simulink library "ASEToolBox2023a"  (R2023a)
settings: Solver=ode45  StartTime=0.0  StopTime=10.0  RelTol=1e-3  EnableMultiTasking=on
values from neighbouring files (symbols this model uses):
  dt = get_param(gcbh, 'g_output_datatype')    [maskSysComCallbacks_Receive.m]    (also in maskSysComCallbacks_Send.m = get_param(gcbh, 'g_input_datatype'))
undefined symbols (not defined in the file or in its folder): dCx, dCy, dCz, DiscIntNeverNeededParam, Discrete, dmassX, dmassY, dmassZ, dMx, dMy, dMz, dp, dp0, dp1, dp2, dp3, lmd_high, lmd_low, magnitude, Newton, p0, p1, p2, p3, p4, phi0, phi000, phi1, phi2, phi3, phi4, r1, r2, r3, r4, Raphson, theta0, theta1, theta2, theta3, theta4, Time, u0, u1, u2, u3, v0, v0_max, v0_min, v1, v111, v2, v222, v3, v333, v4, W1, w1, w2, W2 ... (+2)
libraries: simulink x38, etargetslib x28, simulink_extras x5, slpidlib x2, ctrlSharedLib x2, aerolibatmos2 x1, aerolibconvert2 x1, aerolibtransform2 x1, sharedtransform x1, dspstat3 x1, dspsolvers x1
(part 6 of 6)

== matlab function ASEToolBox2023a/Subsystem/Formation-Control/Consistent formation control /一致性控制——F1/Subsystem1/MATLAB Function ==
  data: i input; wx output; dt input; wy output
function [wx,wy] = w_error(i,dt)
%W_ERROR 此处显示有关此函数的摘要
%   此处显示详细说明
wx = 0.1*(cos(i*dt+pi/6)+cos(i*dt/3+pi/6)+cos(i*dt/5+pi/6)+cos(i*dt/7+pi/6));
wy = 0.1*(sin(i*dt+pi/6)+sin(i*dt/3+pi/6)+sin(i*dt/5+pi/6)+sin(i*dt/7+pi/6));

end

== matlab function ASEToolBox2023a/Subsystem/Formation-Control/Consistent formation control /一致性控制——F2/Subsystem2/MATLAB Function ==
  data: i input; wx output; dt input; wy output
function [wx,wy] = w_error(i,dt)
%W_ERROR 此处显示有关此函数的摘要
%   此处显示详细说明
wx = 0.1*(cos(i*dt+pi/6)+cos(i*dt/3+pi/6)+cos(i*dt/5+pi/6)+cos(i*dt/7+pi/6));
wy = 0.1*(sin(i*dt+pi/6)+sin(i*dt/3+pi/6)+sin(i*dt/5+pi/6)+sin(i*dt/7+pi/6));

end

== matlab function ASEToolBox2023a/Subsystem/Formation-Control/Consistent formation control /一致性控制——F3/Subsystem1/MATLAB Function ==
  data: i input; wx output; dt input; wy output
function [wx,wy] = w_error(i,dt)
%W_ERROR 此处显示有关此函数的摘要
%   此处显示详细说明
wx = 0.1*(cos(i*dt+pi/6)+cos(i*dt/3+pi/6)+cos(i*dt/5+pi/6)+cos(i*dt/7+pi/6));
wy = 0.1*(sin(i*dt+pi/6)+sin(i*dt/3+pi/6)+sin(i*dt/5+pi/6)+sin(i*dt/7+pi/6));

end

== matlab function ASEToolBox2023a/Subsystem/Formation-Control/Follower1/MATLAB Function ==
  data: theta input; J output; phi input; v input
function J = TA_xyz(theta,phi,v)
a=cos(theta)*cos(phi);
b=-v*sin(theta)*cos(phi);
c=-v*cos(theta)*sin(phi);

d=sin(theta)*cos(phi);
e=v*cos(theta)*cos(phi);
f=-v*sin(theta)*sin(phi);

g=sin(phi);
h=0;
i=v*cos(phi);

J=[a,b,c;
    d,e,f;
    g,h,i];
end

== matlab function ASEToolBox2023a/Subsystem/Formation-Control/Consistent formation control /一致性控制——F2/MATLAB Function2 ==
  data: r input; result output
function result = Faixy(r)
%UNTITLED 此处显示有关此函数的摘要


result=-1.8*(1-exp(-0.5*r))/(1+exp(-0.5*r));



end

== matlab function ASEToolBox2023a/Subsystem/Formation-Control/Consistent formation control /一致性控制——F1/MATLAB Function1 ==
  data: r input; result output
function result = Faixy(r)
%UNTITLED 此处显示有关此函数的摘要


result=-1.8*(1-exp(-0.5*r))/(1+exp(-0.5*r));



end

== matlab function ASEToolBox2023a/Subsystem/Formation-Control/Consistent formation control /一致性控制——F1/MATLAB Function2 ==
  data: r input; result output
function result = Faixy(r)
%UNTITLED 此处显示有关此函数的摘要


result=-1.8*(1-exp(-0.5*r))/(1+exp(-0.5*r));



end

== matlab function ASEToolBox2023a/Subsystem/Formation-Control/Consistent formation control /一致性控制——F1/MATLAB Function4 ==
  data: r input; result output
function result = Faixy(r)
%UNTITLED 此处显示有关此函数的摘要


result=-1.8*(1-exp(-0.5*r))/(1+exp(-0.5*r));



end

== matlab function ASEToolBox2023a/Subsystem/Formation-Control/Follower1/MATLAB Function3 ==
  data: r input; result output
function result = Faiv(r)
%UNTITLED 此处显示有关此函数的摘要


result=-0.5*(1-exp(-0.5*r))/(1+exp(-0.5*r));



end

== matlab function ASEToolBox2023a/Subsystem/Formation-Control/Consistent formation control /一致性控制——F3/MATLAB Function3 ==
  data: r input; result output
function result = Faixy(r)
%UNTITLED 此处显示有关此函数的摘要


result=-1.8*(1-exp(-0.5*r))/(1+exp(-0.5*r));



end

== matlab function ASEToolBox2023a/Subsystem/Formation-Control/Follower3/MATLAB Function3 ==
  data: r input; result output
function result = Faiv(r)
%UNTITLED 此处显示有关此函数的摘要


result=-0.5*(1-exp(-0.5*r))/(1+exp(-0.5*r));



end

== matlab function ASEToolBox2023a/Subsystem/Formation-Control/Leader/MATLAB Function ==
  data: theta input; J output; phi input; v input
function J = TA_xyz(theta,phi,v)
a=cos(theta)*cos(phi);
b=-v*sin(theta)*cos(phi);
c=-v*cos(theta)*sin(phi);

d=sin(theta)*cos(phi);
e=v*cos(theta)*cos(phi);
f=-v*sin(theta)*sin(phi);

g=sin(phi);
h=0;
i=v*cos(phi);

J=[a,b,c;
    d,e,f;
    g,h,i];
end

== matlab function ASEToolBox2023a/Subsystem/GNC_EKF/GPS_Data_Process/TD_baro/MATLAB Function2 ==
  data: T input single; u1 output; u0 input; u1 input single; u2 input single; h input single; r input single; u2 output
function [u1,u2]=diff_TD_2(T,u0,u1,u2,h,r)
    %init
    %T是信号周期，u0原始信号输入，u1跟踪原始信号，u2原始信号差分值，
    %h滤波因子（h=T时接近一阶差分）越大滤波好延迟大；r速度因子，越大跟踪的越快但是噪声放大；

x1=0; x2=0;
delta=0;
delta0=0;
y=0;
fabs_y=0;
a0=0;
a=0;
fst=0;

x1 = u1;
x2 = u2;
delta = r*h;
delta0 = delta*h;
y = x1 - u0 + h*x2;
fabs_y = abs(y);   
a0 = sqrt(delta*delta + 8 * r*fabs_y);

if (fabs_y <= delta0)
	a = x2 + y / h;
else
    a = x2 + 0.5*(a0 - delta)*sign(y);
end

if (abs(a) <= delta)
	fst = -r*a / delta;
else
	fst = -r*sign(a);
end
u1 = single(x1 + T*x2); %计算跟踪信号
u2 = single(x2 + T*fst); % 计算微分信号

== matlab function ASEToolBox2023a/Subsystem/Formation-Control/Consistent formation control /一致性控制——F2/MATLAB Function3 ==
  data: r input; result output
function result = Faixy(r)
%UNTITLED 此处显示有关此函数的摘要


result=-1.8*(1-exp(-0.5*r))/(1+exp(-0.5*r));



end

== matlab function ASEToolBox2023a/Subsystem/Formation-Control/Follower2/MATLAB Function ==
  data: theta input; J output; phi input; v input
function J = TA_xyz(theta,phi,v)
a=cos(theta)*cos(phi);
b=-v*sin(theta)*cos(phi);
c=-v*cos(theta)*sin(phi);

d=sin(theta)*cos(phi);
e=v*cos(theta)*cos(phi);
f=-v*sin(theta)*sin(phi);

g=sin(phi);
h=0;
i=v*cos(phi);

J=[a,b,c;
    d,e,f;
    g,h,i];
end

== matlab function ASEToolBox2023a/Subsystem/Formation-Control/Follower1/MATLAB Function2 ==
  data: w input; result output
function result = Faiv(w)
%UNTITLED 此处显示有关此函数的摘要


result=-0.5*(1-exp(-0.5*w))/(1+exp(-0.5*w));



end

== matlab function ASEToolBox2023a/Subsystem/Formation-Control/Follower1/MATLAB Function1 ==
  data: W input; result output
function result = Faiv(W)
%UNTITLED 此处显示有关此函数的摘要


result=-0.5*(1-exp(-0.5*W))/(1+exp(-0.5*W));



end

== matlab function ASEToolBox2023a/Subsystem/GNC_EKF/GPS_Data_Process/LLA2NED/initGPSLLA ==
  data: QGCinitflag input; gpsLLA0_rad output; GPSfixtype input; gps_LLA_rad input; init_GPSLLAflag output; GPSHdop input
function [gpsLLA0_rad,init_GPSLLAflag] = initGPSLLA0(QGCinitflag,GPSfixtype,gps_LLA_rad,GPSHdop)
    persistent initGPSLLAflag;
    persistent gpsLLA0;

    if isempty(initGPSLLAflag)
        initGPSLLAflag = 0;
    end
    if isempty(gpsLLA0)
        %初始GPS未进入定位状态，给定值
%          gpsLLA0 = [28.2/57.3;113/57.3;0];
        gpsLLA0 = zeros(3,1);
    end
    %if (initGPSLLAflag == 0 && GPSfixtype >= 3 && GPSHdop <= 2) || (QGCinitflag == 1 && GPSfixtype >= 3)
    if (initGPSLLAflag == 0 && GPSfixtype >= 1 && GPSHdop <= 5) || (QGCinitflag == 1 && GPSfixtype >= 1)
        % 当GPS第一次初始化位置时，当GPSfixtype >=1 时，自动初始化一次位置，initGPSLLAflag置1
        % 或者是利用QGCinitflag地面站重新修正，不过需要满足GPSfixtype>=1的条件
        gpsLLA0 = gps_LLA_rad;
        initGPSLLAflag = 1;
    end
    gpsLLA0_rad = gpsLLA0;
    init_GPSLLAflag = initGPSLLAflag;
end

== matlab function ASEToolBox2023a/Subsystem/Formation-Control/Follower2/MATLAB Function1 ==
  data: W input; result output
function result = Faiv(W)
%UNTITLED 此处显示有关此函数的摘要


result=-0.5*(1-exp(-0.5*W))/(1+exp(-0.5*W));



end

== matlab function ASEToolBox2023a/Subsystem/Formation-Control/Follower2/MATLAB Function2 ==
  data: w input; result output
function result = Faiv(w)
%UNTITLED 此处显示有关此函数的摘要


result=-0.5*(1-exp(-0.5*w))/(1+exp(-0.5*w));



end

== matlab function ASEToolBox2023a/Subsystem/Formation-Control/Follower2/MATLAB Function3 ==
  data: r input; result output
function result = Faiv(r)
%UNTITLED 此处显示有关此函数的摘要


result=-0.5*(1-exp(-0.5*r))/(1+exp(-0.5*r));



end

== matlab function ASEToolBox2023a/Subsystem/GNC_EKF/GPS_Data_Process/TD_baro1/MATLAB Function2 ==
  data: T input single; u1 output; u0 input; u1 input single; u2 input single; h input single; r input single; u2 output
function [u1,u2]=diff_TD_2(T,u0,u1,u2,h,r)
    %init
    %T是信号周期，u0原始信号输入，u1跟踪原始信号，u2原始信号差分值，
    %h滤波因子（h=T时接近一阶差分）越大滤波好延迟大；r速度因子，越大跟踪的越快但是噪声放大；

x1=0; x2=0;
delta=0;
delta0=0;
y=0;
fabs_y=0;
a0=0;
a=0;
fst=0;

x1 = u1;
x2 = u2;
delta = r*h;
delta0 = delta*h;
y = x1 - u0 + h*x2;
fabs_y = abs(y);   
a0 = sqrt(delta*delta + 8 * r*fabs_y);

if (fabs_y <= delta0)
	a = x2 + y / h;
else
    a = x2 + 0.5*(a0 - delta)*sign(y);
end

if (abs(a) <= delta)
	fst = -r*a / delta;
else
	fst = -r*sign(a);
end
u1 = single(x1 + T*x2); %计算跟踪信号
u2 = single(x2 + T*fst); % 计算微分信号
